simulink model "PMLSM_ControlCore_Block"  (R2026a)
settings: Solver=FixedStepDiscrete  StopTime=1  FixedStep=1e-4
values from neighbouring files (symbols this model uses):
  CPU_Clock = 200e6    (= 200000000)    [PMSLM_Init_Params_MBDL4.m]
  Current_Control_Mode = 2    [init_PMLSM_mil_test_params.m]
  DeadTime_Comp_Enable = 0    [init_PMLSM_mil_test_params.m]
  delay_N = 50    [PMSLM_Init_Params_MBDL4.m]
  DPCC_Ld_Factor = 1    [init_PMLSM_mil_test_params.m]
  DPCC_Lq_Factor = 1    [init_PMLSM_mil_test_params.m]
  DPCC_Psi_Factor = 1    [init_PMLSM_mil_test_params.m]
  DPCC_Rs_Factor = 1    [init_PMLSM_mil_test_params.m]
  DPICC_Ld_Factor = 1    [init_PMLSM_mil_test_params.m]
  DPICC_Lq_Factor = 1    [init_PMLSM_mil_test_params.m]
  Hold_Ticks = 30000    [PMSLM_Init_Params_MBDL4.m]
  Id_Init_Step = Id_Init_Target / Ramp_Ticks    (= 5e-05)    [PMSLM_Init_Params_MBDL4.m]
  Id_Init_Target = 0.5    [PMSLM_Init_Params_MBDL4.m]
  Id_Release_Ramp_Ticks = 2000    [PMSLM_Init_Params_MBDL4.m]
  Iq_fric_run = 0.05    [PMSLM_Init_Params_MBDL4.m]
  Iq_fric_start = 0.40    (= 0.4)    [PMSLM_Init_Params_MBDL4.m]
  Iq_int_limit = 0.10    (= 0.1)    [PMSLM_Init_Params_MBDL4.m]
  Kaw_d = Kaw_q    (= 0.2)    [PMSLM_Init_Params_MBDL4.m]
  Kaw_q = 0.2    [PMSLM_Init_Params_MBDL4.m]
  Kaw_s = 0.4    [PMSLM_Init_Params_MBDL4.m]
  Ki_ACR = ACR_Commissioning_Scale*Ki_ACR_Baseline    (= 2962.5)    [PMSLM_Init_Params_MBDL4.m]    (also in init_PMLSM_mil_test_params.m = Kp_ACR*PMLSM_Rs_ohm/PMLSM_Lq_H)
  Ki_ASR = 0.05    [PMSLM_Init_Params_MBDL4.m]
  Kp_ACR = ACR_Commissioning_Scale*Kp_ACR_Baseline    (= 2.18125)    [PMSLM_Init_Params_MBDL4.m]    (also in init_PMLSM_mil_test_params.m = PMLSM_Lq_H/(4*MIL_AUM3S4_Current_PI_xi^2*MIL_AUM3S4_Current_)
  Kp_ASR = 0.03    [PMSLM_Init_Params_MBDL4.m]
  Kp_pos = 5    [PMSLM_Init_Params_MBDL4.m]
  PICDO_Dhat_Limit_A = 3.0    (= 3)    [init_PMLSM_mil_test_params.m]
  PICDO_Kd = 0.25    [init_PMLSM_mil_test_params.m]
  PICDO_Kx = 1.0    (= 1)    [init_PMLSM_mil_test_params.m]
  PMLSM_deadtime_ratio = PMLSM_deadtime_s * PMLSM_pwm_freq_Hz    (= 0.01)    [init_PMLSM_plant_params.m]
  PMLSM_Ld_H = Ld    (= 0.001745)    [PMSLM_Init_Params_MBDL4.m]    (also in init_PMLSM_plant_params.m)
  PMLSM_Lq_H = Lq    (= 0.001745)    [PMSLM_Init_Params_MBDL4.m]    (also in init_PMLSM_plant_params.m)
  PMLSM_psi_f_Wb = flux    (= 0.141)    [PMSLM_Init_Params_MBDL4.m]    (also in init_PMLSM_plant_params.m)
  PMLSM_Rs_ohm = Rs    (= 2.37)    [PMSLM_Init_Params_MBDL4.m]    (also in init_PMLSM_plant_params.m)
  Pos_deadband = 0.02    [PMSLM_Init_Params_MBDL4.m]
  Ramp_Ticks = 10000    [PMSLM_Init_Params_MBDL4.m]
  Speed_Feedback_Mode = 1    [init_PMLSM_mil_test_params.m]
  Speed_loop_Iq_Limit = Iq_Limit    (= 0.3)    [PMSLM_Init_Params_MBDL4.m]
  Tau_e_mm = 60    [PMSLM_Init_Params_MBDL4.m]
  theta_align_const = 0    [PMSLM_Init_Params_MBDL4.m]
  Theta_Offset_Fine = Simulink.Parameter    [PMSLM_Init_Params_MBDL4.m]
  Ts = 1 / PWM_Freq    (= 0.0001)    [PMSLM_Init_Params_MBDL4.m]
  Ts_ACR = 1e-4    (= 0.0001)    [PMSLM_Init_Params_MBDL4.m]
  Ts_ASR = 1e-3    (= 0.001)    [PMSLM_Init_Params_MBDL4.m]
  Ts_DPICC = 1e-4    (= 0.0001)    [init_PMLSM_mil_test_params.m]
  Udc = 48    [PMSLM_Init_Params_MBDL4.m]    (also in init_PMLSM_mil_test_params.m)
  Uq_Zero_EN = 0：q 轴用正常 PI    [PMSLM_Init_Params_MBDL4.m]
  v_ff_eps = 0.5    [PMSLM_Init_Params_MBDL4.m]
  V_meas_max = 500    [PMSLM_Init_Params_MBDL4.m]
  v_meas_zero_eps = 0.5    [PMSLM_Init_Params_MBDL4.m]
  v_over_eps = 3    [PMSLM_Init_Params_MBDL4.m]
  V_pos_max_mmps = 10    [PMSLM_Init_Params_MBDL4.m]
  v_ref_max = 20    [PMSLM_Init_Params_MBDL4.m]
  v_ref_set_step_dn = v_ref_set_rate_dn * Ts    (= 0.005)    [PMSLM_Init_Params_MBDL4.m]
  v_ref_set_step_up = v_ref_set_rate_up * Ts    (= 0.005)    [PMSLM_Init_Params_MBDL4.m]
  v_ref_zero_eps = 0.2    [PMSLM_Init_Params_MBDL4.m]
  v_stick_off = 3.0    (= 3)    [PMSLM_Init_Params_MBDL4.m]
  v_stick_on = 1.0    (= 1)    [PMSLM_Init_Params_MBDL4.m]
  X_max_hard = 500    [PMSLM_Init_Params_MBDL4.m]
  X_max_soft = 470    [PMSLM_Init_Params_MBDL4.m]
  X_min_hard = -500    [PMSLM_Init_Params_MBDL4.m]
  X_min_soft = -470    [PMSLM_Init_Params_MBDL4.m]
libraries: hdlsllib x13, simulink x11, mcbeeMathTransformLib x2, mcbcontrolslib x1
(part 3 of 3)

== system PMLSM_ControlCore_Block/PMLSM_ControlCore/FOC_Algorithm/DPCC_Current_Controller/PICDO_DPICC_Core/PICDO_Observer/Observer_Diagnostics_Pack ==
  obs_did_meas : Inport
  obs_diq_meas : Inport  Port=2
  obs_di_state_d : Inport  Port=3
  obs_di_state_q : Inport  Port=4
  obs_di_corr_d : Inport  Port=5
  obs_di_corr_q : Inport  Port=6
  obs_err_d : Inport  Port=7
  obs_err_q : Inport  Port=8
  obs_D_corr_d : Inport  Port=9
  obs_D_corr_q : Inport  Port=10
  num_err_d : Inport  Port=11
  num_err_q : Inport  Port=12
  num_di_corr_d : Inport  Port=13
  num_di_corr_q : Inport  Port=14
  num_D_corr_d : Inport  Port=15
  num_D_corr_q : Inport  Port=16
  num_next_did : Inport  Port=17
  num_next_diq : Inport  Port=18
  num_next_Dd : Inport  Port=19
  num_next_Dq : Inport  Port=20
  mux_numeric_check_observer : Mux  Inputs=10
  mux_observer_diag : Mux  Inputs=10
  observer_diag : Outport
  numeric_check_observer : Outport  Port=2
  wires:
  obs_did_meas/1 -> mux_observer_diag/1
  num_err_d/1 -> mux_numeric_check_observer/1
  obs_diq_meas/1 -> mux_observer_diag/2
  num_err_q/1 -> mux_numeric_check_observer/2
  obs_di_state_d/1 -> mux_observer_diag/3
  num_di_corr_d/1 -> mux_numeric_check_observer/3
  obs_di_state_q/1 -> mux_observer_diag/4
  num_di_corr_q/1 -> mux_numeric_check_observer/4
  obs_di_corr_d/1 -> mux_observer_diag/5
  num_D_corr_d/1 -> mux_numeric_check_observer/5
  obs_di_corr_q/1 -> mux_observer_diag/6
  num_D_corr_q/1 -> mux_numeric_check_observer/6
  obs_err_d/1 -> mux_observer_diag/7
  num_next_did/1 -> mux_numeric_check_observer/7
  obs_err_q/1 -> mux_observer_diag/8
  num_next_diq/1 -> mux_numeric_check_observer/8
  obs_D_corr_d/1 -> mux_observer_diag/9
  num_next_Dd/1 -> mux_numeric_check_observer/9
  obs_D_corr_q/1 -> mux_observer_diag/10
  num_next_Dq/1 -> mux_numeric_check_observer/10
  mux_observer_diag/1 -> observer_diag/1
  mux_numeric_check_observer/1 -> numeric_check_observer/1

== system PMLSM_ControlCore_Block/PMLSM_ControlCore/FOC_Algorithm/DPCC_Current_Controller/PICDO_DPICC_Core/PICDO_Observer/Observer_Model_Input_Pack ==
  obs_did_meas : Inport
  obs_diq_meas : Inport  Port=2
  obs_du_prev_d : Inport  Port=3
  obs_du_prev_q : Inport  Port=4
  obs_du_act_d : Inport  Port=5
  obs_du_act_q : Inport  Port=6
  obs_D_state_d : Inport  Port=7
  obs_D_state_q : Inport  Port=8
  obs_err_d : Inport  Port=9
  obs_err_q : Inport  Port=10
  obs_di_state_d : Inport  Port=11
  obs_di_state_q : Inport  Port=12
  obs_we : Inport  Port=13
  observer_model_inputs : Mux  Inputs=13
  model_inputs : Outport
  wires:
  obs_did_meas/1 -> observer_model_inputs/1
  obs_diq_meas/1 -> observer_model_inputs/2
  obs_du_prev_d/1 -> observer_model_inputs/3
  obs_du_prev_q/1 -> observer_model_inputs/4
  obs_du_act_d/1 -> observer_model_inputs/5
  obs_du_act_q/1 -> observer_model_inputs/6
  obs_D_state_d/1 -> observer_model_inputs/7
  obs_D_state_q/1 -> observer_model_inputs/8
  obs_err_d/1 -> observer_model_inputs/9
  obs_err_q/1 -> observer_model_inputs/10
  obs_di_state_d/1 -> observer_model_inputs/11
  obs_di_state_q/1 -> observer_model_inputs/12
  obs_we/1 -> observer_model_inputs/13
  observer_model_inputs/1 -> model_inputs/1

== matlab function PMLSM_ControlCore_Block/PMLSM_ControlCore/FOC_Algorithm/DPCC_Current_Controller/PICDO_DPICC_Core/PICDO_Numeric_Protection/finite_check ==
  data: u input; y output
function y = fcn(u)
%#codegen
y = all(isfinite(u));
end

== matlab function PMLSM_ControlCore_Block/PMLSM_ControlCore/Travel_Safety_Manager ==
  data: v_ref_safe output; x_mm input; travel_fault_latch output; v_ref input; X_max_soft input; X_min_soft input; X_max_hard input; X_min_hard input; travel_fault_latch_z input
function [v_ref_safe, travel_fault_latch] = Travel_Safety_Manager( ...
    x_mm, v_ref, X_max_soft, X_min_soft, X_max_hard, X_min_hard, travel_fault_latch_z)
% PMLSM travel safety manager
% 功能：
% 1. 软限位：只限制继续向越界方向运动，不触发硬关断
% 2. 硬限位：触发 travel_fault_latch，锁存故障
% 3. travel_fault_latch = 1 后，v_ref_safe 强制为 0
% 注意：
% 当前版本没有 fault_reset 输入，硬限位故障一旦触发，
% 只能通过 DSP 复位/重新运行程序清除。
% 速度方向判断死区，单位 mm/s
V_eps = 1.0;

% ---------- 1. 硬限位检测 ----------
hard_hi = (x_mm >= X_max_hard);
hard_lo = (x_mm <= X_min_hard);
hard_fault_raw = hard_hi || hard_lo;

% ---------- 2. 外部锁存 ----------
% 上一拍已经故障，或者当前触发硬限位，则继续保持故障
fault_latch_now = (travel_fault_latch_z > 0.5) || hard_fault_raw;

% ---------- 3. 软限位方向性限制 ----------
right_soft = (x_mm >= X_max_soft);
left_soft  = (x_mm <= X_min_soft);

v_pos_dir = (v_ref >  V_eps);
v_neg_dir = (v_ref < -V_eps);

right_block = right_soft && v_pos_dir;
left_block  = left_soft  && v_neg_dir;

soft_block = right_block || left_block;

% ---------- 4. 输出安全速度 ----------
if fault_latch_now
    v_ref_safe = 0.0;
elseif soft_block
    v_ref_safe = 0.0;
else
    v_ref_safe = v_ref;
end

travel_fault_latch = double(fault_latch_now);
end

== stateflow chart PMLSM_ControlCore_Block/PMLSM_ControlCore/Angle_Init ==
  state IDLE
    entry:
    Angle_Init_EN   = 0;
    Init_Done       = 0;
    id_init_ref     = 0;
    Init_State_Num  = 0;
  note: 固定电角度，缓慢建立 d 轴电流。
  note: 保持固定电角度，让动子吸附稳定。
  state RAMP_ID
    entry:
    Angle_Init_EN   = 1;
    Init_Done       = 0;
    id_init_ref     = 0;
    Init_State_Num  = 1;
    during:
    Angle_Init_EN = 1;
    Init_Done     = 0;
    id_init_ref = id_init_ref + Id_Init_Step;
    if (id_init_ref > Id_Init_Target)
    id_init_ref = Id_Init_Target;
    end
  state HOLD_ALIGN
    entry:
    Angle_Init_EN   = 1;
    Init_Done       = 0;
    id_init_ref     = Id_Init_Target;
    Init_State_Num  = 2;
    during:
    Angle_Init_EN = 1;
    Init_Done     = 0;
    id_init_ref   = Id_Init_Target;
  state RAMP_DOWN_ID
    entry:
    Angle_Init_EN   = 1;
    Init_Done       = 0;
    id_init_ref     = Id_Init_Target;
    Init_State_Num  = 3;
    during:
    Angle_Init_EN = 1;
    Init_Done     = 0;
    id_init_ref = id_init_ref - Id_Init_Target/Id_Release_Ramp_Ticks;
    if (id_init_ref < 0)
    id_init_ref = 0;
    end
    Theta_Offset_auto = theta_offset_mem;
  state DONE
    entry:
    Angle_Init_EN   = 0;
    Init_Done       = 1;
    id_init_ref     = 0;
    Init_State_Num  = 4;
    during:
    Angle_Init_EN = 0;
    Init_Done = 1;
    id_init_ref = 0;
    Init_State_Num = 4;
    Theta_Offset_auto = theta_offset_mem;
  HOLD_ALIGN -> IDLE [order 1] : [Init_Reset > 0.5 || travel_fault_latch > 0.5]
  RAMP_ID -> IDLE [order 1] : [Init_Reset > 0.5 || travel_fault_latch > 0.5]
  (default) -> IDLE
  IDLE -> RAMP_ID : [Init_Start > 0.5 && Init_Reset < 0.5 && travel_fault_latch < 0.5]
  RAMP_ID -> HOLD_ALIGN [order 2] : [after(Ramp_Ticks, tick)]
  RAMP_DOWN_ID -> IDLE [order 2] : [Init_Reset > 0.5 || travel_fault_latch > 0.5]
  DONE -> IDLE : [Init_Reset > 0.5 || travel_fault_latch > 0.5]
  HOLD_ALIGN -> RAMP_DOWN_ID [order 2] : [after(Hold_Ticks, tick)]
      | {x_align_mm_latch = x_mm;
      | theta_offset_mem = mod(theta_align_const - 2*pi*x_align_mm_latch/Tau_e_mm, 2*pi);
      | Theta_Offset_auto = theta_offset_mem;}
  RAMP_DOWN_ID -> DONE [order 1] : [after(Id_Release_Ramp_Ticks, tick)]
  data: Init_Start input; Init_Reset input; travel_fault_latch input; Init_Done output; Init_State_Num output; theta_align_const parameter; Tau_e_mm parameter; Id_Init_Target parameter; Ramp_Ticks parameter; Hold_Ticks parameter; Id_Init_Step parameter; id_init_ref output; Angle_Init_EN output; x_mm input; Theta_Offset_auto output; x_align_mm_latch output; theta_offset_mem local; Id_Release_Ramp_Ticks parameter
